simulink library "lindiPlane_lib"  (R2023b)
settings: Solver=VariableStepAuto  StartTime=0.0  StopTime=10.0  RelTol=1e-3
undefined symbols (not defined in the file or in its folder): DiscIntNeverNeededParam, lindi, lindi_notune
libraries: filters_lib x28, $bdroot x20, simulink x12, ca_lib x2, axes_transformation_lib x1, unit_conversions_lib x1, wpnav_lib x1
(part 2 of 2)

== system lindiPlane_lib/LindiPlane Autopilot/Plane Inner Loop INDI and Control Allocation/Avoid Chattering ==
  u : Inport
  Delta_u : Inport  Port=2
  Avoid Chattering : MATLAB Function  TreatAsAtomicUnit=on
  Unit Delay1 : UnitDelay  SampleTime=-1  HasFrameUpgradeWarning=on
  Delta_u_last : Outport
  wires:
  Avoid Chattering/1(Delta_u) -> Delta_u_last/1
  u/1 -> Avoid Chattering/1(u)
  Unit Delay1/1 -> Avoid Chattering/2("Delta_u ")
  Delta_u/1 -> Unit Delay1/1

== system lindiPlane_lib/LindiPlane Autopilot/Plane Inner Loop INDI and Control Allocation/Collective ailerons decay ==
  Delta u_d : Inport
  u : Inport  Port=2
  Enable : EnablePort
  Add1 : Sum
  Constant2 : Constant  Value=ap.ca.u_d
  Gain : Gain  Gain=-ap.dlc.flapdecay
  MATLAB Function2 : MATLAB Function  TreatAsAtomicUnit=on
  Delta nu_acc_z : Outport  OutputWhenDisabled=reset  InitialOutput=0  VectorParamsAs1DForOutWhenUnconnected=off
  wires:
  Gain/1 -> Delta nu_acc_z/1
  u/1 -> MATLAB Function2/1(u)
  Delta u_d/1 -> Add1/1
  Add1/1 -> MATLAB Function2/2(u_d)
  MATLAB Function2/1(Delta_u_aileron_collective) -> Gain/1
  Constant2/1 -> Add1/2

== system lindiPlane_lib/LindiPlane Autopilot/Plane Inner Loop INDI and Control Allocation/De-activate DLC at high pitch angle errors ==
  Delta_nu_acc_z : Inport
  e_Theta : Inport  Port=2
  Enable : EnablePort
  Constant1 : Constant  Value=ap.dlc.maxptch
  MATLAB Function : MATLAB Function  TreatAsAtomicUnit=on
  rad2deg : unit_conversions_lib/rad2deg
      settings: SourceProductName=LADAC
  Delta_nu_acc_z_out : Outport  OutputWhenDisabled=reset  InitialOutput=0  VectorParamsAs1DForOutWhenUnconnected=off
  wires:
  MATLAB Function/1(Delta_nu_acc_z) -> Delta_nu_acc_z_out/1
  Constant1/1 -> MATLAB Function/2(e_Theta_cutoff)
  Delta_nu_acc_z/1 -> MATLAB Function/1("Delta_nu_acc_z ")
  rad2deg/1 -> MATLAB Function/3(e_Theta)
  e_Theta/1 -> rad2deg/1

== system lindiPlane_lib/LindiPlane Autopilot/Plane Inner Loop INDI and Control Allocation/Delta u_d ==
  u : Inport
  Add5 : Sum  Inputs=+-
  Servo and Sensor Filter Delay : $bdroot/LindiPlane Autopilot/Pitch Angle Controller/Servo and Sensor Filter Delay  SystemSampleTime=-1  VariantActivationTime=update diagram  AllowFlexibleInterface=on  Latency=0  AutoFrameSizeCalculation=off
  Terminator : Terminator
  Terminator1 : Terminator
  Delta_u : Outport  VectorParamsAs1DForOutWhenUnconnected=off
  wires:
  u/1 -> Servo and Sensor Filter Delay/1, Add5/1
  Servo and Sensor Filter Delay/1 -> Add5/2
  Add5/1 -> Delta_u/1
  Servo and Sensor Filter Delay/2 -> Terminator1/1
  Servo and Sensor Filter Delay/3 -> Terminator/1

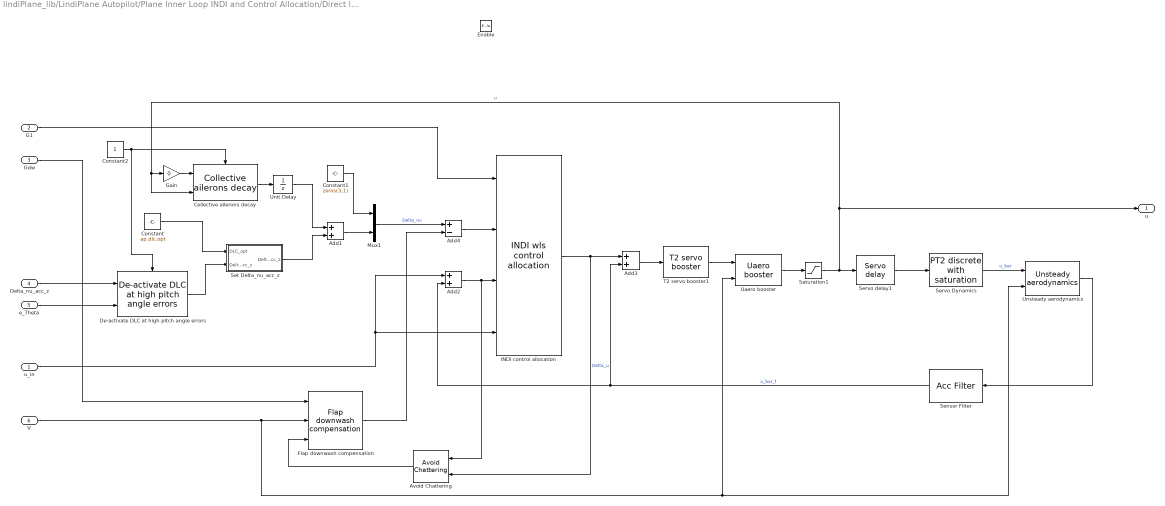
== system lindiPlane_lib/LindiPlane Autopilot/Plane Inner Loop INDI and Control Allocation/Direct lift control - control allocation ==
  u_in : Inport
  G1 : Inport  Port=2
  Gdw : Inport  Port=3
  Delta_nu_acc_z : Inport  Port=4
  e_Theta : Inport  Port=5
  V : Inport  Port=6
  Enable : EnablePort  StatesWhenEnabling=reset
  Add1 : Sum
  Add2 : Sum
  Add3 : Sum
  Add4 : Sum  Inputs=+-
  Avoid Chattering : $bdroot/LindiPlane Autopilot/Plane Inner Loop INDI and Control Allocation/Avoid Chattering  SystemSampleTime=-1  VariantActivationTime=update diagram  AllowFlexibleInterface=on  Latency=0  AutoFrameSizeCalculation=off
  Collective ailerons decay : $bdroot/LindiPlane Autopilot/Plane Inner Loop INDI and Control Allocation/Collective ailerons decay  SystemSampleTime=-1  VariantActivationTime=update diagram  AllowFlexibleInterface=on  Latency=0  AutoFrameSizeCalculation=off
  Constant : Constant  Value=ap.dlc.opt
  Constant1 : Constant  Value=zeros(3,1)
  Constant2 : Constant
  De-activate DLC at high pitch angle errors : $bdroot/LindiPlane Autopilot/Plane Inner Loop INDI and Control Allocation/De-activate DLC at high pitch angle errors  SystemSampleTime=-1  VariantActivationTime=update diagram  AllowFlexibleInterface=on  Latency=0  AutoFrameSizeCalculation=off
  Flap downwash compensation : $bdroot/LindiPlane Autopilot/Plane Inner Loop INDI and Control Allocation/Flap downwash compensation  ceb=ap.ceb  cef=ap.cef  eig=ap.eig
  Gain : Gain  Gain=0
  INDI control allocation : ca_lib/INDI wls control allocation  ca=ap.ca  is_Delta_u_d_checked=on  is_Delta_gamma_checked=off  is_Delta_W_v_checked=off  is_Delta_u_max_checked=off  is_W_checked=off  is_iter_checked=off
      settings: SourceProductName=LADAC
  Mux1 : Mux  Inputs=2
  Saturation1 : Saturate  UpperLimit=ap.ca.u_max  LowerLimit=ap.ca.u_min
  Sensor Filter : $bdroot/LindiPlane Autopilot/Measurement Filtering/Acc Filter  SystemSampleTime=-1  VariantActivationTime=update diagram  AllowFlexibleInterface=on  Latency=0  AutoFrameSizeCalculation=off
  Servo Dynamics : filters_lib/PT2 discrete with saturation  param_src=internal  omega=ap.servo.omega  d=ap.servo.d  x_max=inf  x_min=-inf  x_dt_max=inf  x_dt_min=-inf  x_dt2_max=inf  x_dt2_min=-inf  y_0_src=internal  x_init=0  y_dt_0_src=internal  x_dt_init=0  is_y_dt_checked=off  is_y_dt2_checked=off  is_external_reset_checked=off  mask_expr_handling_config=default
      settings: SourceProductName=LADAC
  Servo delay1 : $bdroot/LindiPlane Autopilot/Plane Inner Loop INDI and Control Allocation/Servo delay  SystemSampleTime=-1  VariantActivationTime=update diagram  AllowFlexibleInterface=on  Latency=0  AutoFrameSizeCalculation=off
  Set Delta_nu_acc_z : MATLAB Function  TreatAsAtomicUnit=on
  T2 servo booster1 : $bdroot/LindiPlane Autopilot/Plane Inner Loop INDI and Control Allocation/T2 servo booster  omega=ap.servo.omega  d=ap.servo.d  b=ap.dlc.srv.boost
  Uaero booster : $bdroot/LindiPlane Autopilot/Plane Inner Loop INDI and Control Allocation/Uaero booster  uaero_use=ap.dlc.ua.use  opt1=ap.dlc.ua.opt1  opt2=ap.dlc.ua.opt2  Vref=ap.dlc.ua.Vref  uaero=ap.uaero  A1=0.165  b1=0.0455  A2=0.335  b2=0.3
  Unit Delay : UnitDelay  SampleTime=-1  HasFrameUpgradeWarning=on
  Unsteady aerodynamics : $bdroot/LindiPlane Autopilot/Plane Inner Loop INDI and Control Allocation/Unsteady aerodynamics  uaero_use=ap.dlc.ua.use
  u : Outport  OutputWhenDisabled=reset  InitialOutput=0  VectorParamsAs1DForOutWhenUnconnected=off
  wires:
  Avoid Chattering/1 -> Flap downwash compensation/3
  Gdw/1 -> Flap downwash compensation/1
  Unit Delay/1 -> Add1/1
  Gain/1 -> Collective ailerons decay/1
  Constant2/1 -> De-activate DLC at high pitch angle errors/Enable, Collective ailerons decay/Enable
  Uaero booster/1 -> Saturation1/1
  Unsteady aerodynamics/1 -> Sensor Filter/1
  V/1 -> Flap downwash compensation/2, Uaero booster/2, Unsteady aerodynamics/2
  Flap downwash compensation/1 -> Add4/2
  Add4/1 -> INDI control allocation/2
  u_in/1 -> Add2/1, INDI control allocation/4
  Collective ailerons decay/1 -> Unit Delay/1
  Add1/1 -> Mux1/2
  Constant1/1 -> Mux1/1
  Mux1/1 -> Add4/1  "Delta_nu"
  Set Delta_nu_acc_z/1(Delta_nu_acc_z) -> Add1/2
  e_Theta/1 -> De-activate DLC at high pitch angle errors/2
  De-activate DLC at high pitch angle errors/1 -> Set Delta_nu_acc_z/2("Delta_nu_acc_z ")
  Delta_nu_acc_z/1 -> De-activate DLC at high pitch angle errors/1
  Constant/1 -> Set Delta_nu_acc_z/1(DLC_opt)
  Saturation1/1 -> Servo delay1/1, u/1, Collective ailerons decay/2, Gain/1  "u"
  Add3/1 -> T2 servo booster1/1
  Sensor Filter/1 -> Add2/2, Add3/2  "u_bar_f"
  Servo delay1/1 -> Servo Dynamics/1
  G1/1 -> INDI control allocation/1
  T2 servo booster1/1 -> Uaero booster/1
  Servo Dynamics/1 -> Unsteady aerodynamics/1  "u_bar"
  INDI control allocation/1 -> Add3/1, Avoid Chattering/2  "Delta_u"
  Add2/1 -> INDI control allocation/3, Avoid Chattering/1

== system lindiPlane_lib/LindiPlane Autopilot/Plane Inner Loop INDI and Control Allocation/Flap downwash compensation ==
  Gdw : Inport
  V : Inport  Port=2
  Delta_u : Inport  Port=3
  Add3 : Sum  Inputs=+-
  Constant1 : Constant  Value=ap.eig.x_h
  Divide : Product  Inputs=*/
  Gdw6 to Gdw4 : MATLAB Function  TreatAsAtomicUnit=on
  MatrixMultiply : Product  Multiplication=Matrix(*)
  PT1 discrete with saturations1 : filters_lib/PT1 discrete with saturations  param_src=external  T=1  x_max=inf  x_min=-inf  x_dt_max=inf  x_dt_min=-inf  y_0_src=internal  x_init=0  is_y_dt_checked=off  is_external_reset_checked=off  mask_expr_handling_config=default
      settings: SourceProductName=LADAC
  Delta_nu_dw : Outport  VectorParamsAs1DForOutWhenUnconnected=off
  wires:
  Gdw6 to Gdw4/1(Gdw4) -> MatrixMultiply/1
  PT1 discrete with saturations1/1 -> Add3/2
  Divide/1 -> PT1 discrete with saturations1/2
  Constant1/1 -> Divide/1
  Add3/1 -> Delta_nu_dw/1
  MatrixMultiply/1 -> Add3/1, PT1 discrete with saturations1/1
  Delta_u/1 -> MatrixMultiply/2
  Gdw/1 -> Gdw6 to Gdw4/1(Gdw6)
  V/1 -> Divide/2

== system lindiPlane_lib/LindiPlane Autopilot/Plane Inner Loop INDI and Control Allocation/Servo delay ==
  u : Inport
  Constant : Constant  Value=ap.servo.delay
  Constant1 : Constant  Value=ap_notune.ts
  Delay{,1..3} (4 alike) : Delay  DelayLength=1  InitialConditionSource=Input port
      settings: InputPortMap=u0,p4
  MATLAB Function : MATLAB Function  TreatAsAtomicUnit=on
  u_delay : Outport  VectorParamsAs1DForOutWhenUnconnected=off
  wires:
  Constant1/1 -> MATLAB Function/7(ts)
  Constant/1 -> MATLAB Function/6(delay)
  Delay/1 -> MATLAB Function/2(u1), Delay1/1
  Delay3/1 -> MATLAB Function/5(u4)
  MATLAB Function/1(u_delay) -> u_delay/1
  Delay2/1 -> MATLAB Function/4(u3), Delay3/1
  Delay1/1 -> Delay2/1, MATLAB Function/3(u2)
  u/1 -> MATLAB Function/1(u0), Delay/1, Delay/2, Delay1/2, Delay2/2, Delay3/2

== system lindiPlane_lib/LindiPlane Autopilot/Plane Inner Loop INDI and Control Allocation/T2 servo booster ==
  u : Inport
  Add2 : Sum  Inputs=+++
  Add3 : Sum  Inputs=+++
  Discrete-Time Integrator1 : DiscreteIntegrator  SampleTime=-1  ICPrevOutput=DiscIntNeverNeededParam  ICPrevScaledInput=DiscIntNeverNeededParam
  Discrete-Time Integrator2 : DiscreteIntegrator  SampleTime=-1  ICPrevOutput=DiscIntNeverNeededParam  ICPrevScaledInput=DiscIntNeverNeededParam
  Gain4 : Gain  Gain=-b*omega*b*omega
  Gain5 : Gain  Gain=-2*d*(b*omega)
  Gain6 : Gain  Gain=(2*d/omega-2*d/(b*omega)/(omega*omega)*b*omega*b*omega)*b*omega*b*omega
  Gain7 : Gain  Gain=b*b
  Gain8 : Gain  Gain=(1-1/(omega*omega)*b*omega*b*omega)*b*omega*b*omega
  u_boost : Outport  VectorParamsAs1DForOutWhenUnconnected=off
  wires:
  Add3/1 -> u_boost/1
  u/1 -> Add2/1, Gain7/1
  Gain8/1 -> Add3/3
  Gain6/1 -> Add3/2
  Gain7/1 -> Add3/1
  Gain4/1 -> Add2/2
  Gain5/1 -> Add2/3
  Discrete-Time Integrator2/1 -> Gain4/1, Gain8/1
  Add2/1 -> Discrete-Time Integrator1/1
  Discrete-Time Integrator1/1 -> Gain5/1, Discrete-Time Integrator2/1, Gain6/1

== system lindiPlane_lib/LindiPlane Autopilot/Plane Inner Loop INDI and Control Allocation/Uaero booster ==
  u : Inport
  V_A : Inport  Port=2
  Compare To Constant : simulink/Logic and Bit Operations/Compare To Constant  relop=>  const=0  OutDataTypeStr=boolean
  Constant : Constant  Value=uaero_use
  Logical Operator : Logic  Operator=NOT  AllPortsSameDT=off  OutDataTypeStr=boolean
  Merge : Merge
  Pass-through : Subsystem
  Uaero booster : Subsystem
  u_boost : Outport  VectorParamsAs1DForOutWhenUnconnected=off
  wires:
  Uaero booster/1(u_boost) -> Merge/2
  V_A/1 -> Uaero booster/2(V_A)
  Pass-through/1(u_out) -> Merge/1
  Merge/1 -> u_boost/1
  Compare To Constant/1 -> Uaero booster/Enable, Logical Operator/1
  Constant/1 -> Compare To Constant/1
  u/1 -> Pass-through/1(u_in), Uaero booster/1(u)
  Logical Operator/1 -> Pass-through/Enable

== system lindiPlane_lib/LindiPlane Autopilot/Plane Inner Loop INDI and Control Allocation/Unsteady aerodynamics ==
  u : Inport
  V : Inport  Port=2
  Compare To Constant : simulink/Logic and Bit Operations/Compare To Constant  relop=>  const=0  OutDataTypeStr=boolean
  Constant : Constant  Value=uaero_use
  Logical Operator : Logic  Operator=NOT  AllPortsSameDT=off  OutDataTypeStr=boolean
  Merge : Merge
  Pass-through : Subsystem
  Unsteady aerodynamics : Subsystem
  u_unst : Outport  VectorParamsAs1DForOutWhenUnconnected=off
  wires:
  Compare To Constant/1 -> Unsteady aerodynamics/Enable, Logical Operator/1
  V/1 -> Unsteady aerodynamics/2(V)
  u/1 -> Pass-through/1(u_in), Unsteady aerodynamics/1(u)
  Unsteady aerodynamics/1(u_unst) -> Merge/2
  Merge/1 -> u_unst/1
  Pass-through/1(u_out) -> Merge/1
  Constant/1 -> Compare To Constant/1
  Logical Operator/1 -> Pass-through/Enable

== system lindiPlane_lib/LindiPlane Autopilot/Plane Inner Loop INDI and Control Allocation/control effectiveness ==
  V : Inport
  rho : Inport  Port=2
  Constant : Constant  Value=ap.ceb.scale
  Display : Display
  Gain : Gain  Gain=0.5
  Product{,1..3,5} (5 alike) : Product
  Square : Math  Operator=square  SignedPower=on
  indiCeFlapFix : MATLAB Function  TreatAsAtomicUnit=on
  G1 : Outport  VectorParamsAs1DForOutWhenUnconnected=off
  Gdw : Outport  Port=2  VectorParamsAs1DForOutWhenUnconnected=off
  wires:
  Product3/1 -> Gdw/1
  Product1/1 -> Product3/2
  indiCeFlapFix/2(Gdw0) -> Product1/1
  Gain/1 -> Product5/2
  rho/1 -> Gain/1
  Constant/1 -> Product2/1, Product3/1
  Product/1 -> Product2/2
  indiCeFlapFix/1(G10) -> Product/1
  Product5/1 -> Product/2, Product1/2
  Square/1 -> Product5/1
  Product2/1 -> Display/1, G1/1
  V/1 -> Square/1

== system lindiPlane_lib/LindiPlane Autopilot/Roll Angle Controller/Feedback Gains ==
  e_Phi : Inport
  p_ref : Inport  Port=2
  p_dt_ref : Inport  Port=3
  p_meas : Inport  Port=4
  p_dt_meas : Inport  Port=5
  Add : Sum  Inputs=3
  Add1 : Sum  Inputs=|+-
  Add2 : Sum  Inputs=|+-
  Gain1 : Gain  Gain=ap.atc.k.rang
  Gain3 : Gain  Gain=ap.atc.k.rrat
  Gain5 : Gain  Gain=ap.atc.k.racc
  nu_cntrl : Outport  VectorParamsAs1DForOutWhenUnconnected=off
  wires:
  Gain1/1 -> Add/1
  e_Phi/1 -> Gain1/1
  Add/1 -> nu_cntrl/1
  Gain3/1 -> Add/2
  Gain5/1 -> Add/3
  p_dt_ref/1 -> Add2/1
  p_ref/1 -> Add1/1
  Add1/1 -> Gain3/1
  Add2/1 -> Gain5/1
  p_meas/1 -> Add1/2
  p_dt_meas/1 -> Add2/2

== system lindiPlane_lib/LindiPlane Autopilot/Roll Angle Controller/Inner Loop Delay Filter ==
  n_g_ref : Inport
  n_g : Inport  Port=2
  x_b_g : Inport  Port=3
  MATLAB Function4 : MATLAB Function  TreatAsAtomicUnit=on
  PT2 Lean Vector1 : filters_lib/PT2 Lean Vector  param_src=internal  omega=2/(2/(ap.servo.omega*ap.servo.boost)+2/ap.sflt.omega)  d=1  x_max=inf  x_min=-inf  x_dt_max=inf  x_dt_min=-inf  x_dt2_max=inf  x_dt2_min=-inf  n_ref_0_src=external  x_init=[0, 0, -1]  n_ref_dt_0_src=internal  x_dt_init=[0, 0, 0]  is_n_dt_checked=on  is_n_dt2_checked=on  is_external_reset_checked=off  mask_expr_handling_config=default
      settings: SourceProductName=LADAC
  e_Phi : Outport
  p_ref : Outport  Port=2
  p_ref_dt : Outport  Port=3
  wires:
  n_g_ref/1 -> PT2 Lean Vector1/1, PT2 Lean Vector1/2
  MATLAB Function4/1(e_Phi) -> e_Phi/1
  MATLAB Function4/2(p_ref) -> p_ref/1
  x_b_g/1 -> MATLAB Function4/4(x_b_g)
  n_g/1 -> MATLAB Function4/5(n_g)
  PT2 Lean Vector1/2 -> MATLAB Function4/2(n_g_ref_dt)
  MATLAB Function4/3(p_ref_dt) -> p_ref_dt/1
  PT2 Lean Vector1/3 -> MATLAB Function4/3(n_g_ref_dt2)
  PT2 Lean Vector1/1 -> MATLAB Function4/1(n_g_ref)  "Phi_ref"

== system lindiPlane_lib/LindiPlane Autopilot/Roll Angle Controller/Lean Vector ==
  M_bg : Inport
  Constant1 : Constant  Value=[1;0;0]  VectorParams1D=off
  MATLAB Function5 : MATLAB Function  TreatAsAtomicUnit=on
  MatrixMultiply : Product  Multiplication=Matrix(*)
  Roll Angle : MATLAB Function  TreatAsAtomicUnit=on
  Transpose : Math  Operator=transpose
  Phi : Outport
  n_g : Outport  Port=2
  x_b_g : Outport  Port=3
  wires:
  Roll Angle/1(Phi) -> Phi/1
  MatrixMultiply/1 -> x_b_g/1
  M_bg/1 -> MATLAB Function5/1(M_bg), Transpose/1, Roll Angle/1(M_bg)
  MATLAB Function5/1(n_g) -> n_g/1
  Constant1/1 -> MatrixMultiply/2
  Transpose/1 -> MatrixMultiply/1

== system lindiPlane_lib/LindiPlane Autopilot/Roll Angle Controller/Reference Model ==
  n_g_des : Inport
  x_b_g : Inport  Port=2
  n_g : Inport  Port=3
  MATLAB Function2 : MATLAB Function  TreatAsAtomicUnit=on
  PT2 Lean Vector : filters_lib/PT2 Lean Vector  param_src=internal  omega=ap.atc.rm.rfreq  d=1  x_max=inf  x_min=-inf  x_dt_max=inf  x_dt_min=-inf  x_dt2_max=inf  x_dt2_min=-inf  n_ref_0_src=external  x_init=[0, 0, -1]  n_ref_dt_0_src=internal  x_dt_init=[0, 0, 0]  is_n_dt_checked=on  is_n_dt2_checked=on  is_external_reset_checked=off  mask_expr_handling_config=default
      settings: SourceProductName=LADAC
  Phi_ref : Outport
  nu_p_dt_ref : Outport  Port=2
  p_ref : Outport  Port=3
  n_g_ref : Outport  Port=4
  wires:
  MATLAB Function2/1(Phi_ref) -> Phi_ref/1
  n_g_des/1 -> PT2 Lean Vector/2, PT2 Lean Vector/1
  PT2 Lean Vector/1 -> MATLAB Function2/1(n_g_ref), n_g_ref/1  "n_g_ref"
  n_g/1 -> MATLAB Function2/5(n_g)
  MATLAB Function2/2(p_ref) -> p_ref/1  "p_ref"
  x_b_g/1 -> MATLAB Function2/4(x_b_g)
  PT2 Lean Vector/2 -> MATLAB Function2/2(n_ref_dt)
  PT2 Lean Vector/3 -> MATLAB Function2/3(n_ref_dt2)
  MATLAB Function2/3(p_ref_dt) -> nu_p_dt_ref/1  "nu_p_dt_ref"

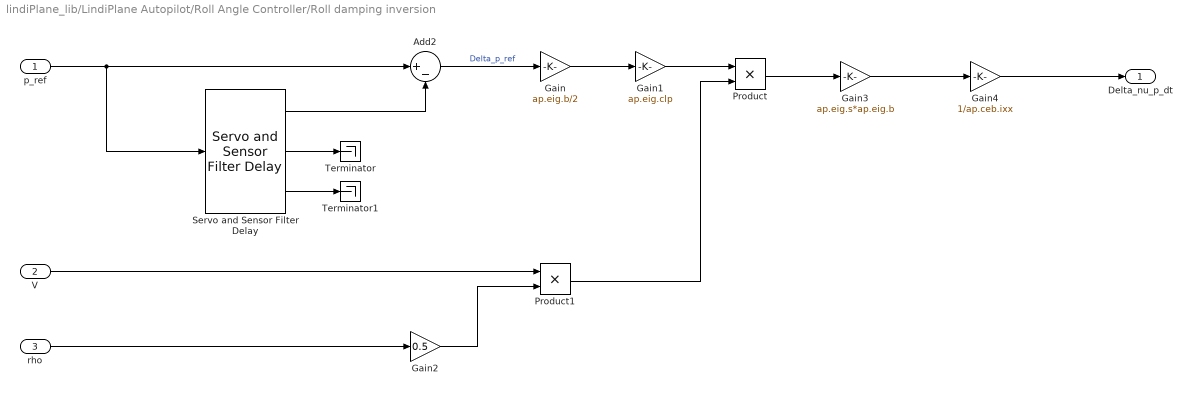
== system lindiPlane_lib/LindiPlane Autopilot/Roll Angle Controller/Roll damping inversion ==
  p_ref : Inport
  V : Inport  Port=2
  rho : Inport  Port=3
  Add2 : Sum  Inputs=|+-
  Gain : Gain  Gain=ap.eig.b/2
  Gain1 : Gain  Gain=ap.eig.clp
  Gain2 : Gain  Gain=0.5
  Gain3 : Gain  Gain=ap.eig.s*ap.eig.b
  Gain4 : Gain  Gain=1/ap.ceb.ixx
  Product : Product
  Product1 : Product
  Servo and Sensor Filter Delay : $bdroot/LindiPlane Autopilot/Pitch Angle Controller/Servo and Sensor Filter Delay  SystemSampleTime=-1  VariantActivationTime=update diagram  AllowFlexibleInterface=on  Latency=0  AutoFrameSizeCalculation=off
  Terminator : Terminator
  Terminator1 : Terminator
  Delta_nu_p_dt : Outport  VectorParamsAs1DForOutWhenUnconnected=off
  wires:
  Servo and Sensor Filter Delay/3 -> Terminator1/1
  Servo and Sensor Filter Delay/2 -> Terminator/1
  Gain4/1 -> Delta_nu_p_dt/1
  Gain3/1 -> Gain4/1
  Product/1 -> Gain3/1
  Product1/1 -> Product/2
  Gain2/1 -> Product1/2
  rho/1 -> Gain2/1
  Gain1/1 -> Product/1
  Gain/1 -> Gain1/1
  Add2/1 -> Gain/1  "Delta_p_ref"
  Servo and Sensor Filter Delay/1 -> Add2/2
  p_ref/1 -> Add2/1, Servo and Sensor Filter Delay/1
  V/1 -> Product1/1

== system lindiPlane_lib/LindiPlane Autopilot/Yaw Rate Controller/Feedback Gains ==
  reference : Inport
  measure : Inport  Port=2
  Add : Sum  Inputs=2
  Add1 : Sum  Inputs=|+-
  Add2 : Sum  Inputs=|+-
  Demux : Demux  Outputs=2
  Demux1 : Demux  Outputs=2
  Gain3 : Gain  Gain=ap.atc.k.yrat
  Gain5 : Gain  Gain=ap.atc.k.yacc
  nu_cntrl : Outport  VectorParamsAs1DForOutWhenUnconnected=off
  wires:
  Add/1 -> nu_cntrl/1
  Gain3/1 -> Add/1
  Gain5/1 -> Add/2
  Demux/2 -> Add2/1
  Demux/1 -> Add1/1
  reference/1 -> Demux/1
  measure/1 -> Demux1/1
  Add1/1 -> Gain3/1
  Add2/1 -> Gain5/1
  Demux1/1 -> Add1/2
  Demux1/2 -> Add2/2

== system lindiPlane_lib/LindiPlane Autopilot/Maneuver Load Alleviation/Maneuver Load Alleviation/Desired Specific Lift ==
  q_ref : Inport
  V_A : Inport  Port=2
  M_bg : Inport  Port=3
  MATLAB Function : MATLAB Function  TreatAsAtomicUnit=on
  a_des_abs : Outport  VectorParamsAs1DForOutWhenUnconnected=off
  wires:
  q_ref/1 -> MATLAB Function/1(q_ref)
  MATLAB Function/1(a_des_abs) -> a_des_abs/1
  V_A/1 -> MATLAB Function/2(V_A)
  M_bg/1 -> MATLAB Function/3(M_bg)

== system lindiPlane_lib/LindiPlane Autopilot/Measurement Filtering/Acc Filter/Subsystem ==
  a_Kb : Inport
  Enable : EnablePort
  T2 Filter (Discrete) : filters_lib/T2 Filter (Discrete)  omega_0=ap.dlc.flt.omega  d=ap.dlc.flt.d  Ts=ap_notune.ts  is_vel=false  is_acc=false  SimulateUsing=Code generation
      settings: SourceProductName=LADAC
  a_Kb_F : Outport  VectorParamsAs1DForOutWhenUnconnected=off
  wires:
  T2 Filter (Discrete)/1 -> a_Kb_F/1  "s_g_f"
  a_Kb/1 -> T2 Filter (Discrete)/1

== system lindiPlane_lib/LindiPlane Autopilot/Measurement Filtering/Acc Filter/Subsystem1 ==
  a_Kb : Inport
  Enable : EnablePort
  T2 Filter (Discrete) : filters_lib/T2 Filter (Discrete)  omega_0=ap.sflt.omega  d=ap.sflt.d  Ts=ap_notune.ts  is_vel=false  is_acc=false  SimulateUsing=Code generation
      settings: SourceProductName=LADAC
  a_Kb_F : Outport  VectorParamsAs1DForOutWhenUnconnected=off
  wires:
  T2 Filter (Discrete)/1 -> a_Kb_F/1  "s_g_f"
  a_Kb/1 -> T2 Filter (Discrete)/1

== system lindiPlane_lib/LindiPlane Autopilot/Pitch Angle Controller/Servo and Sensor Filter Delay/Unsteady Aerodynamics ==
  u : Inport
  Add : Sum  Inputs=+++
  Gain : Gain  Gain=0.5*ap.uaero.fdref
  Uaero 1 : Subsystem  mask{V=ap.uaero.Vref, c=ap.uaero.cref, E=ap.uaero.fdref, A=0.165, b=0.0455, uaero_use=ap.uaero.use, opt=ap.uaero.opt1}
      mask prompts: uaero_use "Use unsteady aerodynamics"; opt "Unsteady aerodynamics boost option"
  Uaero 2 : $bdroot/LindiPlane Autopilot/Pitch Angle Controller/Servo and Sensor Filter Delay/Unsteady Aerodynamics/Uaero 1  V=ap.uaero.Vref  c=ap.uaero.cref  E=ap.uaero.fdref  A=0.335  b=0.3  uaero_use=ap.uaero.use  opt=ap.uaero.opt2
  u_unst : Outport  VectorParamsAs1DForOutWhenUnconnected=off
  wires:
  u/1 -> Gain/1, Uaero 2/1, Uaero 1/1(in)
  Uaero 1/1("out ") -> Add/2
  Uaero 2/1 -> Add/3
  Gain/1 -> Add/1
  Add/1 -> u_unst/1

== system lindiPlane_lib/LindiPlane Autopilot/Pitch Rate Controller/Pitch eigendynamics/Pitch damping ==
  Delta_q_ref : Inport
  V : Inport  Port=2
  rho : Inport  Port=3
  Gain5 : Gain  Gain=ap.eig.x_h
  Gain6 : Gain  Gain=-ap.eig.cla_h
  Gain7 : Gain  Gain=ap.eig.s_h*ap.eig.x_h
  Gain9 : Gain  Gain=0.5
  Product2 : Product
  Product3 : Product
  Delta_M : Outport  VectorParamsAs1DForOutWhenUnconnected=off
  wires:
  rho/1 -> Gain9/1
  Delta_q_ref/1 -> Gain5/1
  Gain5/1 -> Gain6/1
  Gain7/1 -> Delta_M/1
  Product2/1 -> Gain7/1
  Product3/1 -> Product2/2
  V/1 -> Product3/1
  Gain6/1 -> Product2/1
  Gain9/1 -> Product3/2

== system lindiPlane_lib/LindiPlane Autopilot/Pitch Rate Controller/Pitch eigendynamics/Pitch stiffness ==
  Delta_q_ref : Inport
  V : Inport  Port=2
  rho : Inport  Port=3
  Add5 : Sum
  Constant1 : Constant
  Delta angle of attack : Subsystem
  Divide : Product  Inputs=*/
  Downwash transport delay : Subsystem
  Gain1 : Gain  Gain=ap.eig.xnp0-ap.eig.xcg
  Gain12 : Gain  Gain=ap.eig.x_h
  Gain2 : Gain  Gain=ap.eig.xnp-ap.eig.xnp0
  Gain3 : Gain  Gain=ap.ceb.m
  Product1 : Product
  Delta_M : Outport  VectorParamsAs1DForOutWhenUnconnected=off
  wires:
  Gain12/1 -> Downwash transport delay/2(T)
  Gain2/1 -> Downwash transport delay/1(Delta_M)
  Downwash transport delay/1(Delta_M_downwash) -> Add5/2
  Delta angle of attack/1(Delta_alpha) -> Product1/1
  Add5/1 -> Delta_M/1
  V/1 -> Divide/2, Product1/2, Delta angle of attack/2(V)
  Delta_q_ref/1 -> Delta angle of attack/1(Delta_q_ref)  "Delta_q_ref"
  rho/1 -> Delta angle of attack/3(rho)
  Product1/1 -> Gain3/1
  Gain3/1 -> Gain2/1, Gain1/1
  Divide/1 -> Gain12/1
  Constant1/1 -> Divide/1
  Gain1/1 -> Add5/1

== system lindiPlane_lib/LindiPlane Autopilot/Plane Inner Loop INDI and Control Allocation/Uaero booster/Pass-through ==
  u_in : Inport
  Enable : EnablePort
  u_out : Outport  VectorParamsAs1DForOutWhenUnconnected=off
  wires:
  u_in/1 -> u_out/1

== system lindiPlane_lib/LindiPlane Autopilot/Plane Inner Loop INDI and Control Allocation/Uaero booster/Uaero booster ==
  u : Inport
  V_A : Inport  Port=2
  Enable : EnablePort
  Uaero booster1 : Subsystem  mask{opt=opt1, Vref=Vref, uaero=uaero, Aj=A2, bi=b1}
      mask prompts: opt "Option"; Aj "Uaero parameter Aj"; bi "Uaero parameter bi"
  Uaero booster2 : $bdroot/LindiPlane Autopilot/Plane Inner Loop INDI and Control Allocation/Uaero booster/Uaero booster/Uaero booster1  opt=opt2  Vref=Vref  uaero=uaero  Aj=A1  bi=b2
  u_boost : Outport  VectorParamsAs1DForOutWhenUnconnected=off
  wires:
  u/1 -> Uaero booster1/1(u)
  V_A/1 -> Uaero booster1/2(V_A), Uaero booster2/2
  Uaero booster2/1 -> u_boost/1
  Uaero booster1/1(u_boost) -> Uaero booster2/1

== system lindiPlane_lib/LindiPlane Autopilot/Plane Inner Loop INDI and Control Allocation/Unsteady aerodynamics/Pass-through ==
  u_in : Inport
  Enable : EnablePort
  u_out : Outport  VectorParamsAs1DForOutWhenUnconnected=off
  wires:
  u_in/1 -> u_out/1

== system lindiPlane_lib/LindiPlane Autopilot/Plane Inner Loop INDI and Control Allocation/Unsteady aerodynamics/Unsteady aerodynamics ==
  u : Inport
  V : Inport  Port=2
  Enable : EnablePort
  Constant : Constant  Value=ap.uaero.c  VectorParams1D=off
  Constant1 : Constant  Value=ap.uaero.fdepth  VectorParams1D=off
  Constant2 : Constant
  Discrete-Time Integrator : DiscreteIntegrator  InitialConditionSource=external  SampleTime=-1  ICPrevOutput=DiscIntNeverNeededParam  ICPrevScaledInput=DiscIntNeverNeededParam
  Divide : Product  Inputs=*/
  MATLAB Function : MATLAB Function  TreatAsAtomicUnit=on
  MATLAB Function1 : MATLAB Function  TreatAsAtomicUnit=on
  Reshape : Reshape  OutputDimensionality=Row vector (2-D)
  Reshape1 : Reshape
  u_unst : Outport  VectorParamsAs1DForOutWhenUnconnected=off
  wires:
  Discrete-Time Integrator/1 -> MATLAB Function/5(x)
  MATLAB Function/1(c_L_flap) -> Divide/1
  Constant/1 -> MATLAB Function/2(c)
  Reshape1/1 -> u_unst/1
  Constant2/1 -> MATLAB Function/3(C_L_alpha)
  Constant1/1 -> MATLAB Function/4(E)
  MATLAB Function1/1(x0) -> Discrete-Time Integrator/2
  Divide/1 -> Reshape1/1
  MATLAB Function/3(x_dt) -> Discrete-Time Integrator/1
  Reshape/1 -> MATLAB Function/6(eta), MATLAB Function1/1(alpha)
  u/1 -> Reshape/1
  MATLAB Function/2(alpha_deta) -> Divide/2
  V/1 -> MATLAB Function/1(V)

== system lindiPlane_lib/LindiPlane Autopilot/Pitch Angle Controller/Servo and Sensor Filter Delay/Unsteady Aerodynamics/Uaero 1 ==
  in : Inport
  Compare To Constant3 : simulink/Logic and Bit Operations/Compare To Constant  relop=>  const=0  OutDataTypeStr=boolean
  Compare To Constant4 : simulink/Logic and Bit Operations/Compare To Constant  relop=<  const=2  OutDataTypeStr=boolean
  Constant2 : Constant  Value=uaero_use
  Constant3 : Constant  Value=opt
  Gain1 : Gain  Gain=(2-E)*A
  Logical Operator1 : Logic  Operator=NOT  AllPortsSameDT=off  OutDataTypeStr=boolean
  Logical Operator3 : Logic  AllPortsSameDT=off  OutDataTypeStr=boolean
  Merge : Merge
  Pass-through : Subsystem
  Time Delay : Subsystem
  "out " : Outport  VectorParamsAs1DForOutWhenUnconnected=off
  wires:
  in/1 -> Gain1/1
  Gain1/1 -> Pass-through/1(In1), Time Delay/1(In1)
  Time Delay/1(Out1) -> Merge/2
  Pass-through/1(Out1) -> Merge/1
  Merge/1 -> "out "/1
  Logical Operator3/1 -> Time Delay/Enable, Logical Operator1/1
  Constant2/1 -> Compare To Constant3/1
  Constant3/1 -> Compare To Constant4/1
  Compare To Constant3/1 -> Logical Operator3/1
  Compare To Constant4/1 -> Logical Operator3/2
  Logical Operator1/1 -> Pass-through/Enable

== system lindiPlane_lib/LindiPlane Autopilot/Pitch Rate Controller/Pitch eigendynamics/Pitch stiffness/Delta angle of attack ==
  note: In case of ap.dlc.opt=2, the time constant should ideally be zero.
      | However, the time delay of the load factor is currently only halfed by ap.dlc.opt=2.
  Delta_q_ref : Inport
  V : Inport  Port=2
  rho : Inport  Port=3
  Angle of attack time delay : MATLAB Function  TreatAsAtomicUnit=on
  Constant : Constant  Value=ap.dlc.opt
  Constant6 : Constant  Value=ap.ceb.m
  Constant7 : Constant  Value=ap.eig.s
  Constant8 : Constant  Value=ap.eig.cla_h
  Gain : Gain  Gain=0.5
  PT1 discrete with saturations : filters_lib/PT1 discrete with saturations  param_src=external  T=1  x_max=inf  x_min=-inf  x_dt_max=inf  x_dt_min=-inf  y_0_src=internal  x_init=0  is_y_dt_checked=off  is_external_reset_checked=off  mask_expr_handling_config=default
      settings: SourceProductName=LADAC
  Switch : Switch  Criteria=u2 > Threshold  Threshold=1.5  SaturateOnIntegerOverflow=off  InputSameDT=off
  Delta_alpha : Outport  VectorParamsAs1DForOutWhenUnconnected=off
  wires:
  Switch/1 -> PT1 discrete with saturations/2
  Gain/1 -> Switch/1
  Constant/1 -> Switch/2
  Constant6/1 -> Angle of attack time delay/2(m)
  V/1 -> Angle of attack time delay/1(V)
  Constant7/1 -> Angle of attack time delay/4(S)
  Constant8/1 -> Angle of attack time delay/5(C_La)
  rho/1 -> Angle of attack time delay/3(rho)
  Angle of attack time delay/1(T) -> Gain/1, Switch/3
  Delta_q_ref/1 -> PT1 discrete with saturations/1
  PT1 discrete with saturations/1 -> Delta_alpha/1

== system lindiPlane_lib/LindiPlane Autopilot/Pitch Rate Controller/Pitch eigendynamics/Pitch stiffness/Downwash transport delay ==
  Delta_M : Inport
  T : Inport  Port=2
  Gain : Gain  Gain=0.5
  PT1 discrete with saturations : filters_lib/PT1 discrete with saturations  param_src=external  T=1  x_max=inf  x_min=-inf  x_dt_max=inf  x_dt_min=-inf  y_0_src=internal  x_init=0  is_y_dt_checked=off  is_external_reset_checked=off  mask_expr_handling_config=default
      settings: SourceProductName=LADAC
  PT1 discrete with saturations1 : filters_lib/PT1 discrete with saturations  param_src=external  T=1  x_max=inf  x_min=-inf  x_dt_max=inf  x_dt_min=-inf  y_0_src=internal  x_init=0  is_y_dt_checked=off  is_external_reset_checked=off  mask_expr_handling_config=default
      settings: SourceProductName=LADAC
  Delta_M_downwash : Outport  VectorParamsAs1DForOutWhenUnconnected=off
  wires:
  Delta_M/1 -> PT1 discrete with saturations/1
  PT1 discrete with saturations/1 -> PT1 discrete with saturations1/1
  PT1 discrete with saturations1/1 -> Delta_M_downwash/1
  T/1 -> Gain/1
  Gain/1 -> PT1 discrete with saturations1/2, PT1 discrete with saturations/2

== system lindiPlane_lib/LindiPlane Autopilot/Plane Inner Loop INDI and Control Allocation/Uaero booster/Uaero booster/Uaero booster1 ==
  u : Inport
  V_A : Inport  Port=2
  Compare To Constant1 : simulink/Logic and Bit Operations/Compare To Constant  relop===  const=1  OutDataTypeStr=boolean
  Compare To Constant2 : simulink/Logic and Bit Operations/Compare To Constant  relop===  const=0  OutDataTypeStr=boolean
  Constant : Constant  Value=opt
  Eliminate Uaero i : Subsystem
  Logical Operator : Logic  Operator=NOT  AllPortsSameDT=off  OutDataTypeStr=boolean
  Logical Operator1 : Logic  Operator=NOT  AllPortsSameDT=off  OutDataTypeStr=boolean
  Merge : Merge
  Merge1 : Merge
  Pass-through : Subsystem
  Uaero Inversion i : Subsystem  mask{uaero=uaero, Aj=Aj, bi=bi}
  Uaero Reference i : Subsystem  mask{E=uaero.fdref, c=uaero.cref, V=uaero.Vref, Aj=Aj, bi=bi}
      mask prompts: E "Eref"; c "cref"; V "Vref"
  u_boost : Outport  VectorParamsAs1DForOutWhenUnconnected=off
  wires:
  Logical Operator1/1 -> Uaero Inversion i/Enable
  Compare To Constant2/1 -> Pass-through/Enable, Logical Operator1/1
  Merge1/1 -> u_boost/1
  Pass-through/1(u_ref) -> Merge1/1
  V_A/1 -> Uaero Inversion i/2(V_A)
  Merge/1 -> Pass-through/1(u), Uaero Inversion i/1(u)
  Constant/1 -> Compare To Constant1/1, Compare To Constant2/1
  Eliminate Uaero i/1(u_ref) -> Merge/1
  Uaero Reference i/1(u_boost) -> Merge/2
  Logical Operator/1 -> Eliminate Uaero i/Enable
  u/1 -> Uaero Reference i/1(u), Eliminate Uaero i/1(u)
  Compare To Constant1/1 -> Logical Operator/1, Uaero Reference i/Enable
  Uaero Inversion i/1(u_boost) -> Merge1/2

== system lindiPlane_lib/LindiPlane Autopilot/Pitch Angle Controller/Servo and Sensor Filter Delay/Unsteady Aerodynamics/Uaero 1/Pass-through ==
  In1 : Inport
  Enable : EnablePort
  Out1 : Outport  VectorParamsAs1DForOutWhenUnconnected=off
  wires:
  In1/1 -> Out1/1

== system lindiPlane_lib/LindiPlane Autopilot/Pitch Angle Controller/Servo and Sensor Filter Delay/Unsteady Aerodynamics/Uaero 1/Time Delay ==
  In1 : Inport
  Enable : EnablePort
  Add : Sum  Inputs=+-
  Discrete-Time Integrator : DiscreteIntegrator  InitialConditionSource=external  SampleTime=-1  ICPrevOutput=DiscIntNeverNeededParam  ICPrevScaledInput=DiscIntNeverNeededParam
  Gain : Gain  Gain=2*V*b/c
  Out1 : Outport  VectorParamsAs1DForOutWhenUnconnected=off
  wires:
  Gain/1 -> Discrete-Time Integrator/1
  In1/1 -> Discrete-Time Integrator/2, Add/1
  Add/1 -> Gain/1
  Discrete-Time Integrator/1 -> Out1/1, Add/2

== system lindiPlane_lib/LindiPlane Autopilot/Plane Inner Loop INDI and Control Allocation/Uaero booster/Uaero booster/Uaero booster1/Eliminate Uaero i ==
  u : Inport
  Enable : EnablePort
  u_ref : Outport  VectorParamsAs1DForOutWhenUnconnected=off
  wires:
  u/1 -> u_ref/1

== system lindiPlane_lib/LindiPlane Autopilot/Plane Inner Loop INDI and Control Allocation/Uaero booster/Uaero booster/Uaero booster1/Pass-through ==
  u : Inport
  Enable : EnablePort
  u_ref : Outport  VectorParamsAs1DForOutWhenUnconnected=off
  wires:
  u/1 -> u_ref/1

== system lindiPlane_lib/LindiPlane Autopilot/Plane Inner Loop INDI and Control Allocation/Uaero booster/Uaero booster/Uaero booster1/Uaero Inversion i ==
  u : Inport
  V_A : Inport  Port=2
  Enable : EnablePort
  Add : Sum
  Add1 : Sum
  Constant : Constant  Value=uaero.fdepth
  Constant1 : Constant  Value=uaero.c
  Discrete-Time Integrator : DiscreteIntegrator  SampleTime=-1  ICPrevOutput=DiscIntNeverNeededParam  ICPrevScaledInput=DiscIntNeverNeededParam
  Gain2 : Gain
  Product : Product
  Product1 : Product
  Product2 : Product
  State-Space Model Parameters : MATLAB Function  TreatAsAtomicUnit=on
  u_boost : Outport  VectorParamsAs1DForOutWhenUnconnected=off
  wires:
  Constant1/1 -> State-Space Model Parameters/3(c)
  Constant/1 -> State-Space Model Parameters/2(E)
  State-Space Model Parameters/3(D) -> Product2/1
  State-Space Model Parameters/1(A) -> Product1/2
  State-Space Model Parameters/2(B) -> Product/2
  V_A/1 -> State-Space Model Parameters/1(V_A)
  Product2/1 -> Add1/1
  Add1/1 -> u_boost/1
  Gain2/1 -> Add1/2
  Product/1 -> Add/1
  Product1/1 -> Add/2
  Add/1 -> Discrete-Time Integrator/1
  Discrete-Time Integrator/1 -> Gain2/1, Product1/1
  u/1 -> Product/1, Product2/2

== system lindiPlane_lib/LindiPlane Autopilot/Plane Inner Loop INDI and Control Allocation/Uaero booster/Uaero booster/Uaero booster1/Uaero Reference i ==
  u : Inport
  Enable : EnablePort
  Add : Sum
  Add1 : Sum
  Discrete-Time Integrator : DiscreteIntegrator  SampleTime=-1  ICPrevOutput=DiscIntNeverNeededParam  ICPrevScaledInput=DiscIntNeverNeededParam
  Gain2 : Gain
  Product : Product
  Product1 : Product
  Product2 : Product
  State-Space Model Parameters : MATLAB Function  TreatAsAtomicUnit=on
  u_boost : Outport  VectorParamsAs1DForOutWhenUnconnected=off
  wires:
  u/1 -> Product2/2, Product/1
  Discrete-Time Integrator/1 -> Product1/1, Gain2/1
  Add/1 -> Discrete-Time Integrator/1
  Product1/1 -> Add/2
  Product/1 -> Add/1
  Gain2/1 -> Add1/2
  Add1/1 -> u_boost/1
  Product2/1 -> Add1/1
  State-Space Model Parameters/2(B) -> Product/2
  State-Space Model Parameters/1(A) -> Product1/2
  State-Space Model Parameters/3(D) -> Product2/1

== matlab function lindiPlane_lib/LindiPlane Autopilot/Plane Inner Loop INDI and Control Allocation/De-activate DLC at high pitch angle errors/MATLAB Function ==
  data: Delta_nu_acc_z input; e_Theta_cutoff input; Delta_nu_acc_z output; e_Theta input
function Delta_nu_acc_z = fcn(Delta_nu_acc_z, e_Theta_cutoff, e_Theta)
Delta_nu_acc_z(:) = exp(-(0.9124/e_Theta_cutoff*abs(e_Theta)).^4) * Delta_nu_acc_z;
end

== matlab function lindiPlane_lib/LindiPlane Autopilot/Plane Inner Loop INDI and Control Allocation/Direct lift control - control allocation/Set Delta_nu_acc_z ==
  data: DLC_opt input; Delta_nu_acc_z input; Delta_nu_acc_z output
function Delta_nu_acc_z = fcn(DLC_opt, Delta_nu_acc_z)
if DLC_opt < 1.5
    Delta_nu_acc_z(:) = 0;
end
end

== matlab function lindiPlane_lib/LindiPlane Autopilot/Plane Inner Loop INDI and Control Allocation/Flap downwash compensation/Gdw6 to Gdw4 ==
  data: Gdw6 input; Gdw4 output
function Gdw4 = fcn(Gdw6)
Gdw4 = Gdw6([1,2,3,6],:);
end

== matlab function lindiPlane_lib/LindiPlane Autopilot/Plane Inner Loop INDI and Control Allocation/Only rotational control effectiveness ==
  data: G input; G4xX output; DLC_opt input
function G4xX = fcn(G, DLC_opt)
G4xX = G([1:3,6],:);
% avoid collective aileron deflection
if DLC_opt == 0
    G4xX(2,1:end-2) = 0;
    G4xX(4,:) = 0;
end
end

== matlab function lindiPlane_lib/LindiPlane Autopilot/Plane Inner Loop INDI and Control Allocation/Servo delay/MATLAB Function ==
  data: u0 input; u1 input; u2 input; u3 input; u4 input; u_delay output; delay input; ts input
function u_delay = fcn(u0,u1,u2,u3,u4,delay,ts)
num_delays = floor( divideFinite( delay, ts ) );
num_delays(:) = min( num_delays, 4 );
num_delays(:) = max( num_delays, 0 );
if num_delays == 0
    u_delay = u0;
elseif num_delays == 1
    u_delay = u1;
elseif num_delays == 2
    u_delay = u2;
elseif num_delays == 3
    u_delay = u3;
else
    u_delay = u4;
end
end

== matlab function lindiPlane_lib/LindiPlane Autopilot/Plane Inner Loop INDI and Control Allocation/Uaero booster/Uaero booster/Uaero booster1/Uaero Inversion i/State-Space Model Parameters ==
  data: V_A input; A output; B output; D output; Aj parameter; bi parameter; E input; c input
function [A,B,D] = fcn(V_A, Aj, bi, E, c)

% Time constant
Ti = c/(2*V_A*bi);

% Transfer function parameters
b1 = Ti;
b0 = 1;
a1 = 0.5*E.*Ti+(2-E)*Aj.*Ti;
a0 = 1;

% State-space model parameters
A = -a0./a1;
B = 1./a1.*(b0-a0*b1./a1);
D = b1./a1;

end

== matlab function lindiPlane_lib/LindiPlane Autopilot/Plane Inner Loop INDI and Control Allocation/Uaero booster/Uaero booster/Uaero booster1/Uaero Reference i/State-Space Model Parameters ==
  data: V parameter; A output; B output; D output; E parameter; c parameter; Aj parameter; bi parameter
function [A,B,D] = fcn(V, E, c, Aj, bi)

% Time constant
Ti = c/(2*V*bi);

% Transfer function parameters
b1 = 0.5*E.*Ti+(2-E)*Aj.*Ti;
b0 = 1;
a1 = Ti;
a0 = 1;

% State-space model parameters
A = -a0./a1;
B = 1./a1.*(b0-a0*b1./a1);
D = b1./a1;

end

== matlab function lindiPlane_lib/LindiPlane Autopilot/Plane Inner Loop INDI and Control Allocation/Unsteady aerodynamics/Unsteady aerodynamics/MATLAB Function ==
  data: V input; c_L_flap output; alpha_deta output; c input; C_L_alpha input; E input; x input; x_dt output; eta input
function [c_L_flap,alpha_deta,x_dt] = airfoilFlapWagner( V, c, C_L_alpha, E, x, eta )
[c_L_flap,alpha_deta,x_dt] = airfoilFlapWagner( V, c, C_L_alpha, E, x, eta );
end

== matlab function lindiPlane_lib/LindiPlane Autopilot/Plane Inner Loop INDI and Control Allocation/Unsteady aerodynamics/Unsteady aerodynamics/MATLAB Function1 ==
  data: alpha input; x0 output
function x0 = fcn(alpha)
x0 = zeros(2,length(alpha),class(alpha));
end

== matlab function lindiPlane_lib/LindiPlane Autopilot/Plane Inner Loop INDI and Control Allocation/control effectiveness/indiCeFlapFix ==
  data: G10 output; cef parameter; ceb parameter; Gdw0 output; eig parameter
function [G10,Gdw0] = indiCeFlapFix( cef, ceb, eig )
[G10,Gdw0] = indiCeFlapFix( cef, ceb, eig );
end

== matlab function lindiPlane_lib/LindiPlane Autopilot/Roll Angle Controller/Desired Roll Angle ==
  data: x_b_g input; Phi_des output; n_g_des input
function Phi_des  = fcn(x_b_g, n_g_des)
y_b_des_g = cross( x_b_g, n_g_des );
M_bg = [ x_b_g'; y_b_des_g'; -n_g_des' ];
Phi_des = atan2( M_bg(2,3), M_bg(3,3) ); % see dcm2Euler
end

== matlab function lindiPlane_lib/LindiPlane Autopilot/Rudder Decay Controller/Rudder command ==
  data: u input; y output
function y = fcn(u)

y = u(end-1);

== matlab function lindiPlane_lib/LindiPlane Autopilot/Turn Coordination/Turn Coordination ==
  data: Phi input; q output; V input; r output
function [q,r] = fcn(Phi,V)
if abs(Phi) > 0.8*pi/2
    Phi = sign(Phi)*0.8*pi/2;
end
a = 9.81 * tan(Phi);
if V < 1
    V(:) = 1;
end
omega = a/V;
q = omega * sin(Phi);
r = omega * cos(Phi);
end

== matlab function lindiPlane_lib/LindiPlane Autopilot/Roll Angle Controller/Lean Vector/MATLAB Function5 ==
  data: M_bg input; n_g output
function n_g = dcm2LeanVector(M_bg)
n_g = dcm2LeanVector(M_bg);
end

== matlab function lindiPlane_lib/LindiPlane Autopilot/Roll Angle Controller/Lean Vector/Roll Angle ==
  data: M_bg input; Phi output
function Phi = fcn(M_bg)
Phi = atan2( M_bg(2,3), M_bg(3,3) ); % see dcm2Euler
end

== matlab function lindiPlane_lib/LindiPlane Autopilot/Cmd 2 Lean Vector/Cmd Roll 2 n_g_cmd ==
  data: Phi_cmd input; n_g_cmd output; M_bg input
function n_g_cmd = fcn(Phi_cmd, M_bg)
EulerAngles = dcm2Euler(M_bg);
EulerAngles(1) = Phi_cmd;
M_bg = euler2Dcm(EulerAngles);
n_g_cmd = dcm2LeanVector(M_bg);
end

== matlab function lindiPlane_lib/LindiPlane Autopilot/Roll Angle Controller/Reference Model/MATLAB Function2 ==
  data: n_g_ref input; Phi_ref output; n_ref_dt input; n_ref_dt2 input; x_b_g input; p_ref output; n_g input; p_ref_dt output
function [Phi_ref,p_ref,p_ref_dt] = fcn(n_g_ref,n_ref_dt, n_ref_dt2, x_b_g, n_g)
y_b_g = cross( x_b_g, n_g );
p_ref = dot( y_b_g, n_ref_dt );
p_ref_dt = dot( y_b_g, n_ref_dt2 );
% Auxilliary output: Phi_ref
y_b_ref_g = cross( x_b_g, n_g_ref );
M_bg = [ x_b_g'; y_b_ref_g'; -n_g_ref' ];
Phi_ref = atan2( M_bg(2,3), M_bg(3,3) ); % see dcm2Euler
end

== matlab function lindiPlane_lib/LindiPlane Autopilot/Roll Angle Controller/Inner Loop Delay Filter/MATLAB Function4 ==
  data: n_g_ref input; n_g_ref_dt input; n_g_ref_dt2 input; e_Phi output; x_b_g input; p_ref output; n_g input; p_ref_dt output
function [e_Phi,p_ref,p_ref_dt] = fcn(n_g_ref, n_g_ref_dt, n_g_ref_dt2, x_b_g, n_g)
y_b_g = cross( x_b_g, n_g );
e_Phi = atan2(dot(n_g_ref,y_b_g),dot(n_g_ref,n_g));
p_ref = dot( y_b_g, n_g_ref_dt );
p_ref_dt = dot( y_b_g, n_g_ref_dt2 );
end

== matlab function lindiPlane_lib/LindiPlane Autopilot/Maneuver Load Alleviation/Maneuver Load Alleviation/Desired Specific Lift/MATLAB Function ==
  data: q_ref input; a_des_abs output; V_A input; M_bg input
function a_des_abs = fcn(q_ref, V_A, M_bg)
g_b = M_bg*[0;0;9.81];
a_des_abs = q_ref*V_A + g_b(3);
end

== matlab function lindiPlane_lib/LindiPlane Autopilot/Maneuver Load Alleviation/Maneuver Load Alleviation/Maneuver Load Alleviation ==
  data: G10 input; nu_a_Kz input; y_cp_flap input; Delta_u_d output size=size(ap.cef.y); y_np_wing input; ca_main parameter; ca_mla parameter; G11 output; Delta_nu output
function [Delta_u_d,G11,Delta_nu] = fcn(G10,nu_a_Kz,y_cp_flap, y_np_wing,ca_main, ca_mla)
num_flaps = int32(length(y_cp_flap)-2);
Delta_u_d = zeros(1,num_flaps+2,class(nu_a_Kz));

u = zeros(num_flaps+1,1,class(nu_a_Kz));

ca.u_min = ca_main.u_min(1:num_flaps+1);
ca.u_max = ca_main.u_max(1:num_flaps+1);
ca.u_d = ca_main.u_d(1:num_flaps+1);
ca.W_v = ca_mla.W_v;
ca.W_u = ca_mla.W_u(1:num_flaps+1);
ca.gamma = ca_mla.gamma;
ca.W = ca_main.W(1:num_flaps+1);
ca.i_max = ca_mla.i_max;

G11_1 = zeros(1,num_flaps+1,class(nu_a_Kz));
G11_2 = zeros(1,num_flaps+1,class(nu_a_Kz));
G11_1(1:num_flaps/2) = -G10(6,1:num_flaps/2).*abs(y_cp_flap(1:num_flaps/2));
G11_2(num_flaps/2+1:num_flaps) = -G10(6,num_flaps/2+1:num_flaps).*abs(y_cp_flap(num_flaps/2+1:num_flaps));
G11 = [G11_1;G11_2;G10(2,1:num_flaps+1);G10(6,1:num_flaps+1)];

% Pull-up maneuver load alleviation
wrbm = abs(y_np_wing) * nu_a_Kz/2;


% Delta_u_d(1:8) = pinv(G11) * [wrbm(:);0];
Delta_nu = [ wrbm(:); 0; 0 ];
Delta_u_d(1:num_flaps+1) = caIndiWls( ca, G11, Delta_nu, u );

end

== matlab function lindiPlane_lib/LindiPlane Autopilot/Outer Loop INDI/Outer Loop INDI ==
  data: n_g_des output; nu_a_Kb_yz input; Delta_q output; Delta_r output; V input; M_bg input; a_Kg input; n_g_des_last input; Delta_Phi_comp input; q_des output; r_des output; a_abs_des output; a_abs output
function [ n_g_des, Delta_q, Delta_r, q_des, r_des, a_abs_des, a_abs ] = ...
    indiPlaneAcc2LeanQR( nu_a_Kb_yz, V, M_bg, a_Kg, n_g_des_last, Delta_Phi_comp )
    [ n_g_des, Delta_q, Delta_r, q_des, r_des, a_abs_des, a_abs ] = ...
        indiPlaneAcc2LeanQR( nu_a_Kb_yz, V, M_bg, a_Kg, n_g_des_last, Delta_Phi_comp );
end

== matlab function lindiPlane_lib/LindiPlane Autopilot/Pitch Rate Controller/Pitch eigendynamics/Pitch stiffness/Delta angle of attack/Angle of attack time delay ==
  data: V input; T output; m input; rho input; S input; C_La input
function T = fcn(V,m,rho,S,C_La)
A_alpha = divideFinite(V,m)*rho/2*S*C_La;
T = divideFinite( 1, A_alpha );
end

== matlab function lindiPlane_lib/LindiPlane Autopilot/Plane Inner Loop INDI and Control Allocation/Avoid Chattering/Avoid Chattering ==
  data: u input; Delta_u output; Delta_u input; ap parameter
function Delta_u = fcn(u, Delta_u, ap)
% If elevator signal is close to saturation, there will be chattering in
% the control inputs when using the flap downwash high-pass filter. That is
% why we disable the flap downwash high-pass filter if we are close to
% saturation.
u_max = ap.ca.u_max(end-1);
u_min = ap.ca.u_min(end-1);
u_range = u_max - u_min;
if u(end-1) > u_max - 0.1*u_range || u(end-1) < u_min + 0.1*u_range
    Delta_u(:) = 0;
end
end

== matlab function lindiPlane_lib/LindiPlane Autopilot/Plane Inner Loop INDI and Control Allocation/Collective ailerons decay/MATLAB Function2 ==
  data: u input; Delta_u_aileron_collective output; u_d input
function Delta_u_aileron_collective = fcn(u, u_d)
Delta_u_aileron_collective = mean(u_d(1:end-2)-u(1:end-2));
end
